simulink model "MOBATSim"  (R2020b)
settings: Solver=FixedStepAuto  StartTime=0.0  StopTime=Sim_t  FixedStep=0.01  MinStep=0.01  RelTol=1e-2
values from neighbouring files (symbols this model uses):
  Vehicles = evalin('base','Vehicles')    [I2V.m]    (also in VehicleSensors.m)
undefined symbols (not defined in the file or in its folder): Sim_Ts
libraries: simulink x50, robotalgslib x10, drivingvehiclecontroller x10, mpcadaslib x10, pid_lib x10
(part 4 of 7)

== system MOBATSim/Vehicle Model 6/Vehicle Model/Kinematic Bicycle Model ==
  v : Inport
  Steering Angle : Inport  Port=2
  Cos : Trigonometry  Operator=cos
  Gain : Gain  Gain=1/3
  Mux : Mux  Inputs=3
  Mux1 : Mux  Inputs=3
  Product : Product
  Product1 : Product
  Product2 : Product
  Saturation : Saturate  UpperLimit=pi/4  LowerLimit=-pi/4
  Sin : Trigonometry
  Tan : Trigonometry  Operator=tan
  theta : Integrator  InitialCondition=Vehicles(Vehicle_id).dynamics.orientation(4)
  x : Integrator  InitialCondition=Vehicles(Vehicle_id).dynamics.position(1)
  y : Integrator  InitialCondition=-Vehicles(Vehicle_id).dynamics.position(3)
  state : Outport
  stateDot : Outport  Port=2
  wires:
  Tan/1 -> Product2/2
  Product1/1 -> Mux1/2, y/1
  theta/1 -> Cos/1, Sin/1, Mux/3
  v/1 -> Gain/1, Product1/1, Product/1
  Gain/1 -> Product2/1
  Product/1 -> Mux1/1, x/1
  Mux/1 -> state/1
  Sin/1 -> Product1/2
  Steering Angle/1 -> Saturation/1
  Cos/1 -> Product/2
  Product2/1 -> Mux1/3, theta/1
  y/1 -> Mux/2
  x/1 -> Mux/1
  Mux1/1 -> stateDot/1
  Saturation/1 -> Tan/1

== system MOBATSim/Vehicle Model 7/Longitudinal and Lateral Controllers/Lateral Motion Control ==
  note: 1) Add Subsystem or Model blocks as valid variant choices.
      | 2) You cannot connect blocks at this level. At simulation, connectivity is automatically
      | determined, based on the active variant and port name matching.
  speed : Inport
  pose : Inport  Port=2
  changeLane : Inport  Port=3
  Pure Pursuit : Subsystem  VariantControl=PURE_PURSUIT
  Stanley : Subsystem  VariantControl=STANLEY
  SteerCmd : Outport

== system MOBATSim/Vehicle Model 7/Longitudinal and Lateral Controllers/Longitudinal Speed Control ==
  note: The vehicle calculates the speed difference between the actual speed and the reference speed, then generates the acceleration command accordingly.
  Speed Reference : Inport
  Inter Vehicular Distance : Inport  Port=2
  Lead Speed : Inport  Port=3
  Driving Mode : Inport  Port=4
  Dist2Stop : Inport  Port=5
  Actual Speed : Inport  Port=6
  Distance to Stop Controller1 : Subsystem
  Longitudinal Distance Control : Subsystem  Variant=on  VariantControlMode=label  LabelModeActiveChoice=MPC-based  mask{VehicleFollowingControl=MPC-based}
      mask prompts: VehicleFollowingControl "Vehicle Following Control"
      mask TypeOptions VehicleFollowingControl: PID-based | MPC-based
      mask Callback VehicleFollowingControl: set_param(gcb,'OverrideUsingVariant',get_param(gcb,'VehicleFollowingControl'));
      mask Display: image('MOBATSIM-Icon-Set-11 - Platoon.png'); % Use "Edit Image" on toolstrip to change.
  Reference Acceleration Generation : Subsystem
  Reference speed according to the driving mode : Subsystem
  Signal Specification1 : SignalSpecification  Dimensions=1
  Sum13 : Sum  Inputs=|+-
  Longitduinal Acceleration Command : Outport  VectorParamsAs1DForOutWhenUnconnected=off
  wires:
  Longitudinal Distance Control/1(Reference Speed) -> Reference speed according to the driving mode/3(2)
  Lead Speed/1 -> Longitudinal Distance Control/2(Lead Speed)
  Driving Mode/1 -> Reference Acceleration Generation/1(Driving Mode), Reference speed according to the driving mode/1(Driving Mode)
  Signal Specification1/1 -> Longitduinal Acceleration Command/1
  Sum13/1 -> Reference Acceleration Generation/2(Speed Error)
  Inter Vehicular Distance/1 -> Longitudinal Distance Control/1(Relative distance)
  Dist2Stop/1 -> Distance to Stop Controller1/1(Distance to Stop)
  Speed Reference/1 -> Reference speed according to the driving mode/2(1)
  Distance to Stop Controller1/1(ref speed) -> Reference speed according to the driving mode/4(4)
  Reference Acceleration Generation/1(Reference Acceleration Command) -> Signal Specification1/1
  Actual Speed/1 -> Longitudinal Distance Control/3(Ego Speed), Reference Acceleration Generation/3(Actual Speed), Sum13/2
  Reference speed according to the driving mode/1(Reference Speed) -> Sum13/1

== system MOBATSim/Vehicle Model 7/Path Planner/Astar ==
  CommunicationIDs : Inport
  Path Planner - AStar : MATLABSystem  System=VehiclePathPlanner_Astar  Vehicle_id=Vehicle_id  SimulateUsing=Interpreted execution
      mask Type: VehiclePathPlanner_Astar
      mask Display:
      | image('MOBATSIM-Icon-Set_8- Navigation.png');
      | port_label('input',1,'CommunicationIDs');
      | port_label('output',1,'waypointReached');
  waypointReached : Outport
  wires:
  CommunicationIDs/1 -> Path Planner - AStar/1
  Path Planner - AStar/1 -> waypointReached/1

== system MOBATSim/Vehicle Model 7/Path Planner/ShortestPathFinder ==
  CommunicationIDs : Inport
  Path Planner - Shortest : MATLABSystem  System=VehiclePathPlanner_shortestPathFinder  Vehicle_id=Vehicle_id  SimulateUsing=Interpreted execution
      mask Type: VehiclePathPlanner_shortestPathFinder
      mask Display:
      | image('MOBATSIM-Icon-Set_8- Navigation.png');
      | port_label('input',1,'CommunicationIDs');
      | port_label('output',1,'waypointReached');
  waypointReached : Outport
  wires:
  Path Planner - Shortest/1 -> waypointReached/1
  CommunicationIDs/1 -> Path Planner - Shortest/1

== system MOBATSim/Vehicle Model 7/Vehicle Model/Kinematic Bicycle Model ==
  v : Inport
  Steering Angle : Inport  Port=2
  Cos : Trigonometry  Operator=cos
  Gain : Gain  Gain=1/3
  Mux : Mux  Inputs=3
  Mux1 : Mux  Inputs=3
  Product : Product
  Product1 : Product
  Product2 : Product
  Saturation : Saturate  UpperLimit=pi/4  LowerLimit=-pi/4
  Sin : Trigonometry
  Tan : Trigonometry  Operator=tan
  theta : Integrator  InitialCondition=Vehicles(Vehicle_id).dynamics.orientation(4)
  x : Integrator  InitialCondition=Vehicles(Vehicle_id).dynamics.position(1)
  y : Integrator  InitialCondition=-Vehicles(Vehicle_id).dynamics.position(3)
  state : Outport
  stateDot : Outport  Port=2
  wires:
  Tan/1 -> Product2/2
  Product1/1 -> Mux1/2, y/1
  theta/1 -> Cos/1, Sin/1, Mux/3
  v/1 -> Gain/1, Product1/1, Product/1
  Gain/1 -> Product2/1
  Product/1 -> Mux1/1, x/1
  Mux/1 -> state/1
  Sin/1 -> Product1/2
  Steering Angle/1 -> Saturation/1
  Cos/1 -> Product/2
  Product2/1 -> Mux1/3, theta/1
  y/1 -> Mux/2
  x/1 -> Mux/1
  Mux1/1 -> stateDot/1
  Saturation/1 -> Tan/1

== system MOBATSim/Vehicle Model 8/Longitudinal and Lateral Controllers/Lateral Motion Control ==
  note: 1) Add Subsystem or Model blocks as valid variant choices.
      | 2) You cannot connect blocks at this level. At simulation, connectivity is automatically
      | determined, based on the active variant and port name matching.
  speed : Inport
  pose : Inport  Port=2
  changeLane : Inport  Port=3
  Pure Pursuit : Subsystem  VariantControl=PURE_PURSUIT
  Stanley : Subsystem  VariantControl=STANLEY
  SteerCmd : Outport

== system MOBATSim/Vehicle Model 8/Longitudinal and Lateral Controllers/Longitudinal Speed Control ==
  note: The vehicle calculates the speed difference between the actual speed and the reference speed, then generates the acceleration command accordingly.
  Speed Reference : Inport
  Inter Vehicular Distance : Inport  Port=2
  Lead Speed : Inport  Port=3
  Driving Mode : Inport  Port=4
  Dist2Stop : Inport  Port=5
  Actual Speed : Inport  Port=6
  Distance to Stop Controller1 : Subsystem
  Longitudinal Distance Control : Subsystem  Variant=on  VariantControlMode=label  LabelModeActiveChoice=MPC-based  mask{VehicleFollowingControl=MPC-based}
      mask prompts: VehicleFollowingControl "Vehicle Following Control"
      mask TypeOptions VehicleFollowingControl: PID-based | MPC-based
      mask Callback VehicleFollowingControl: set_param(gcb,'OverrideUsingVariant',get_param(gcb,'VehicleFollowingControl'));
      mask Display: image('MOBATSIM-Icon-Set-11 - Platoon.png'); % Use "Edit Image" on toolstrip to change.
  Reference Acceleration Generation : Subsystem
  Reference speed according to the driving mode : Subsystem
  Signal Specification1 : SignalSpecification  Dimensions=1
  Sum13 : Sum  Inputs=|+-
  Longitduinal Acceleration Command : Outport  VectorParamsAs1DForOutWhenUnconnected=off
  wires:
  Longitudinal Distance Control/1(Reference Speed) -> Reference speed according to the driving mode/3(2)
  Lead Speed/1 -> Longitudinal Distance Control/2(Lead Speed)
  Driving Mode/1 -> Reference Acceleration Generation/1(Driving Mode), Reference speed according to the driving mode/1(Driving Mode)
  Signal Specification1/1 -> Longitduinal Acceleration Command/1
  Sum13/1 -> Reference Acceleration Generation/2(Speed Error)
  Inter Vehicular Distance/1 -> Longitudinal Distance Control/1(Relative distance)
  Dist2Stop/1 -> Distance to Stop Controller1/1(Distance to Stop)
  Speed Reference/1 -> Reference speed according to the driving mode/2(1)
  Distance to Stop Controller1/1(ref speed) -> Reference speed according to the driving mode/4(4)
  Reference Acceleration Generation/1(Reference Acceleration Command) -> Signal Specification1/1
  Actual Speed/1 -> Longitudinal Distance Control/3(Ego Speed), Reference Acceleration Generation/3(Actual Speed), Sum13/2
  Reference speed according to the driving mode/1(Reference Speed) -> Sum13/1

== system MOBATSim/Vehicle Model 8/Path Planner/Astar ==
  CommunicationIDs : Inport
  Path Planner - AStar : MATLABSystem  System=VehiclePathPlanner_Astar  Vehicle_id=Vehicle_id  SimulateUsing=Interpreted execution
      mask Type: VehiclePathPlanner_Astar
      mask Display:
      | image('MOBATSIM-Icon-Set_8- Navigation.png');
      | port_label('input',1,'CommunicationIDs');
      | port_label('output',1,'waypointReached');
  waypointReached : Outport
  wires:
  CommunicationIDs/1 -> Path Planner - AStar/1
  Path Planner - AStar/1 -> waypointReached/1

== system MOBATSim/Vehicle Model 8/Path Planner/ShortestPathFinder ==
  CommunicationIDs : Inport
  Path Planner - Shortest : MATLABSystem  System=VehiclePathPlanner_shortestPathFinder  Vehicle_id=Vehicle_id  SimulateUsing=Interpreted execution
      mask Type: VehiclePathPlanner_shortestPathFinder
      mask Display:
      | image('MOBATSIM-Icon-Set_8- Navigation.png');
      | port_label('input',1,'CommunicationIDs');
      | port_label('output',1,'waypointReached');
  waypointReached : Outport
  wires:
  Path Planner - Shortest/1 -> waypointReached/1
  CommunicationIDs/1 -> Path Planner - Shortest/1

== system MOBATSim/Vehicle Model 8/Vehicle Model/Kinematic Bicycle Model ==
  v : Inport
  Steering Angle : Inport  Port=2
  Cos : Trigonometry  Operator=cos
  Gain : Gain  Gain=1/3
  Mux : Mux  Inputs=3
  Mux1 : Mux  Inputs=3
  Product : Product
  Product1 : Product
  Product2 : Product
  Saturation : Saturate  UpperLimit=pi/4  LowerLimit=-pi/4
  Sin : Trigonometry
  Tan : Trigonometry  Operator=tan
  theta : Integrator  InitialCondition=Vehicles(Vehicle_id).dynamics.orientation(4)
  x : Integrator  InitialCondition=Vehicles(Vehicle_id).dynamics.position(1)
  y : Integrator  InitialCondition=-Vehicles(Vehicle_id).dynamics.position(3)
  state : Outport
  stateDot : Outport  Port=2
  wires:
  Tan/1 -> Product2/2
  Product1/1 -> Mux1/2, y/1
  theta/1 -> Cos/1, Sin/1, Mux/3
  v/1 -> Gain/1, Product1/1, Product/1
  Gain/1 -> Product2/1
  Product/1 -> Mux1/1, x/1
  Mux/1 -> state/1
  Sin/1 -> Product1/2
  Steering Angle/1 -> Saturation/1
  Cos/1 -> Product/2
  Product2/1 -> Mux1/3, theta/1
  y/1 -> Mux/2
  x/1 -> Mux/1
  Mux1/1 -> stateDot/1
  Saturation/1 -> Tan/1

== system MOBATSim/Vehicle Model 9/Longitudinal and Lateral Controllers/Lateral Motion Control ==
  note: 1) Add Subsystem or Model blocks as valid variant choices.
      | 2) You cannot connect blocks at this level. At simulation, connectivity is automatically
      | determined, based on the active variant and port name matching.
  speed : Inport
  pose : Inport  Port=2
  changeLane : Inport  Port=3
  Pure Pursuit : Subsystem  VariantControl=PURE_PURSUIT
  Stanley : Subsystem  VariantControl=STANLEY
  SteerCmd : Outport

== system MOBATSim/Vehicle Model 9/Longitudinal and Lateral Controllers/Longitudinal Speed Control ==
  note: The vehicle calculates the speed difference between the actual speed and the reference speed, then generates the acceleration command accordingly.
  Speed Reference : Inport
  Inter Vehicular Distance : Inport  Port=2
  Lead Speed : Inport  Port=3
  Driving Mode : Inport  Port=4
  Dist2Stop : Inport  Port=5
  Actual Speed : Inport  Port=6
  Distance to Stop Controller1 : Subsystem
  Longitudinal Distance Control : Subsystem  Variant=on  VariantControlMode=label  LabelModeActiveChoice=MPC-based  mask{VehicleFollowingControl=MPC-based}
      mask prompts: VehicleFollowingControl "Vehicle Following Control"
      mask TypeOptions VehicleFollowingControl: PID-based | MPC-based
      mask Callback VehicleFollowingControl: set_param(gcb,'OverrideUsingVariant',get_param(gcb,'VehicleFollowingControl'));
      mask Display: image('MOBATSIM-Icon-Set-11 - Platoon.png'); % Use "Edit Image" on toolstrip to change.
  Reference Acceleration Generation : Subsystem
  Reference speed according to the driving mode : Subsystem
  Signal Specification1 : SignalSpecification  Dimensions=1
  Sum13 : Sum  Inputs=|+-
  Longitduinal Acceleration Command : Outport  VectorParamsAs1DForOutWhenUnconnected=off
  wires:
  Longitudinal Distance Control/1(Reference Speed) -> Reference speed according to the driving mode/3(2)
  Lead Speed/1 -> Longitudinal Distance Control/2(Lead Speed)
  Driving Mode/1 -> Reference Acceleration Generation/1(Driving Mode), Reference speed according to the driving mode/1(Driving Mode)
  Signal Specification1/1 -> Longitduinal Acceleration Command/1
  Sum13/1 -> Reference Acceleration Generation/2(Speed Error)
  Inter Vehicular Distance/1 -> Longitudinal Distance Control/1(Relative distance)
  Dist2Stop/1 -> Distance to Stop Controller1/1(Distance to Stop)
  Speed Reference/1 -> Reference speed according to the driving mode/2(1)
  Distance to Stop Controller1/1(ref speed) -> Reference speed according to the driving mode/4(4)
  Reference Acceleration Generation/1(Reference Acceleration Command) -> Signal Specification1/1
  Actual Speed/1 -> Longitudinal Distance Control/3(Ego Speed), Reference Acceleration Generation/3(Actual Speed), Sum13/2
  Reference speed according to the driving mode/1(Reference Speed) -> Sum13/1

== system MOBATSim/Vehicle Model 9/Path Planner/Astar ==
  CommunicationIDs : Inport
  Path Planner - AStar : MATLABSystem  System=VehiclePathPlanner_Astar  Vehicle_id=Vehicle_id  SimulateUsing=Interpreted execution
      mask Type: VehiclePathPlanner_Astar
      mask Display:
      | image('MOBATSIM-Icon-Set_8- Navigation.png');
      | port_label('input',1,'CommunicationIDs');
      | port_label('output',1,'waypointReached');
  waypointReached : Outport
  wires:
  CommunicationIDs/1 -> Path Planner - AStar/1
  Path Planner - AStar/1 -> waypointReached/1

== system MOBATSim/Vehicle Model 9/Path Planner/ShortestPathFinder ==
  CommunicationIDs : Inport
  Path Planner - Shortest : MATLABSystem  System=VehiclePathPlanner_shortestPathFinder  Vehicle_id=Vehicle_id  SimulateUsing=Interpreted execution
      mask Type: VehiclePathPlanner_shortestPathFinder
      mask Display:
      | image('MOBATSIM-Icon-Set_8- Navigation.png');
      | port_label('input',1,'CommunicationIDs');
      | port_label('output',1,'waypointReached');
  waypointReached : Outport
  wires:
  Path Planner - Shortest/1 -> waypointReached/1
  CommunicationIDs/1 -> Path Planner - Shortest/1

== system MOBATSim/Vehicle Model 9/Vehicle Model/Kinematic Bicycle Model ==
  v : Inport
  Steering Angle : Inport  Port=2
  Cos : Trigonometry  Operator=cos
  Gain : Gain  Gain=1/3
  Mux : Mux  Inputs=3
  Mux1 : Mux  Inputs=3
  Product : Product
  Product1 : Product
  Product2 : Product
  Saturation : Saturate  UpperLimit=pi/4  LowerLimit=-pi/4
  Sin : Trigonometry
  Tan : Trigonometry  Operator=tan
  theta : Integrator  InitialCondition=Vehicles(Vehicle_id).dynamics.orientation(4)
  x : Integrator  InitialCondition=Vehicles(Vehicle_id).dynamics.position(1)
  y : Integrator  InitialCondition=-Vehicles(Vehicle_id).dynamics.position(3)
  state : Outport
  stateDot : Outport  Port=2
  wires:
  Tan/1 -> Product2/2
  Product1/1 -> Mux1/2, y/1
  theta/1 -> Cos/1, Sin/1, Mux/3
  v/1 -> Gain/1, Product1/1, Product/1
  Gain/1 -> Product2/1
  Product/1 -> Mux1/1, x/1
  Mux/1 -> state/1
  Sin/1 -> Product1/2
  Steering Angle/1 -> Saturation/1
  Cos/1 -> Product/2
  Product2/1 -> Mux1/3, theta/1
  y/1 -> Mux/2
  x/1 -> Mux/1
  Mux1/1 -> stateDot/1
  Saturation/1 -> Tan/1

== system MOBATSim/Vehicle Model 1/Longitudinal and Lateral Controllers/Lateral Motion Control/Pure Pursuit ==
  pose : Inport
  speed : Inport  Port=2
  changeLane : Inport  Port=3
  MATLAB System : MATLABSystem  System=PurePursuit_WPGenerator  Vehicle_id=Vehicle_id  SimulateUsing=Interpreted execution
      mask Type: PurePursuit_WPGenerator
      mask Display:
      | image('MOBATSIM-Icon-Set_9- PurePursuit WP Generator.png');
      | port_label('input',1,'pose');
      | port_label('input',2,'speed');
      | port_label('input',3,'changeLane');
      | port_label('output',1,'nextWPs');
  Pure Pursuit : robotalgslib/Pure Pursuit  DesiredLinearVelocity=Vehicles(Vehicle_id).dynamics.maxSpeed  MaxAngularVelocity=1  LookaheadDistance=6  TargetDirPort=on  SimulateUsing=Code generation
  Terminator : Terminator
  Terminator1 : Terminator
  Wheel Steering Angle Formulation : Subsystem
  SteerCmd : Outport
  wires:
  MATLAB System/1 -> Pure Pursuit/2
  pose/1 -> Pure Pursuit/1, MATLAB System/1
  speed/1 -> MATLAB System/2
  changeLane/1 -> MATLAB System/3
  Pure Pursuit/3 -> Wheel Steering Angle Formulation/1(alpha)
  Pure Pursuit/1 -> Terminator/1
  Pure Pursuit/2 -> Terminator1/1
  Wheel Steering Angle Formulation/1(referenceYawAngle) -> SteerCmd/1

== system MOBATSim/Vehicle Model 1/Longitudinal and Lateral Controllers/Lateral Motion Control/Stanley ==
  pose : Inport
  speed : Inport  Port=2
  changeLane : Inport  Port=3
  Constant5 : Constant
  Deg to Rad : Gain  Gain=pi/180
  Lateral Controller Stanley : drivingvehiclecontroller/Lateral Controller Stanley  ModelType=Kinematic bicycle model  PositionGainF=2.5  PositionGainR=2.5  YawRateGain=0.2  DelayGain=0.2  VehicleMass=1575  Lf=1.2  Lr=1.6  TireStiffness=19000  Wheelbase=3  MaxSteeringAngle=35
      settings: SourceProductBaseCode=DR
  Stanley Reference Pose Generator : MATLABSystem  System=Stanley_RefPoseGenerator  Vehicle_id=Vehicle_id  SimulateUsing=Interpreted execution
      mask Type: Stanley_RefPoseGenerator
      mask Display:
      | image('MOBATSIM-Icon-Set_10- Stanley.png');
      | port_label('input',1,'pose');
      | port_label('input',2,'speed');
      | port_label('input',3,'changeLane');
      | port_label('output',1,'poseOut');
      | port_label('output',2,'referencePose');
  SteerCmd : Outport
  wires:
  Constant5/1 -> Lateral Controller Stanley/4
  Lateral Controller Stanley/1 -> Deg to Rad/1
  changeLane/1 -> Stanley Reference Pose Generator/3
  Stanley Reference Pose Generator/1 -> Lateral Controller Stanley/2
  Stanley Reference Pose Generator/2 -> Lateral Controller Stanley/1
  pose/1 -> Stanley Reference Pose Generator/1
  speed/1 -> Lateral Controller Stanley/3, Stanley Reference Pose Generator/2
  Deg to Rad/1 -> SteerCmd/1

== system MOBATSim/Vehicle Model 1/Longitudinal and Lateral Controllers/Longitudinal Speed Control/Distance to Stop Controller1 ==
  Distance to Stop : Inport
  Compare To Constant : simulink/Logic and Bit Operations/Compare To Constant  relop=>=  const=10  OutDataTypeStr=uint8
  Gain : Gain  Gain=0.08
  Product : Product
  ref speed : Outport  VectorParamsAs1DForOutWhenUnconnected=off
  wires:
  Distance to Stop/1 -> Compare To Constant/1, Gain/1
  Gain/1 -> Product/1
  Compare To Constant/1 -> Product/2
  Product/1 -> ref speed/1

== system MOBATSim/Vehicle Model 1/Longitudinal and Lateral Controllers/Longitudinal Speed Control/Longitudinal Distance Control ==
  note: 1) Add Subsystem or Model blocks as valid variant choices.
      | 2) You cannot connect blocks at this level. At simulation, connectivity is automatically
      | determined, based on the active variant and port name matching.
  Relative distance : Inport
  Lead Speed : Inport  Port=2
  Ego Speed : Inport  Port=3
  MPC-based : Subsystem  VariantControl=MPC-based
  PID-based : Subsystem  VariantControl=PID-based
  Reference Speed : Outport

== system MOBATSim/Vehicle Model 1/Longitudinal and Lateral Controllers/Longitudinal Speed Control/Reference Acceleration Generation ==
  Driving Mode : Inport
  Speed Error : Inport  Port=2
  Actual Speed : Inport  Port=3
  Emergency Brake : Constant  Value=Vehicles(Vehicle_id).dynamics.minDeceleration
  Multiport Switch3 : MultiPortSwitch  Inputs=4
  Saturation Dynamic : simulink/Discontinuities/Saturation Dynamic  OutMin=[]  OutMax=[]  OutDataTypeStr=Inherit: Same as second input  OutDataType=fixdt(1, 16)  OutScaling=2^-10  DoSatur=off
  Simple Gear Logic : MATLAB Function  TreatAsAtomicUnit=on
  Reference Acceleration Command : Outport  VectorParamsAs1DForOutWhenUnconnected=off
  wires:
  Driving Mode/1 -> Multiport Switch3/1
  Speed Error/1 -> Saturation Dynamic/2
  Emergency Brake/1 -> Saturation Dynamic/3, Multiport Switch3/4
  Saturation Dynamic/1 -> Multiport Switch3/5, Multiport Switch3/2, Multiport Switch3/3
  Actual Speed/1 -> Simple Gear Logic/1(speed)
  Multiport Switch3/1 -> Reference Acceleration Command/1
  Simple Gear Logic/1(maxAcc) -> Saturation Dynamic/1

== system MOBATSim/Vehicle Model 1/Longitudinal and Lateral Controllers/Longitudinal Speed Control/Reference speed according to the driving mode ==
  Driving Mode : Inport
  1 : Inport  Port=2
  2 : Inport  Port=3
  4 : Inport  Port=4
  Constant1 : Constant  Value=0
  Max Speed : Saturate  UpperLimit=Vehicles(Vehicle_id).dynamics.maxSpeed  LowerLimit=-100
  Multiport Switch : MultiPortSwitch  Inputs=4
  Reference Speed : Outport
  wires:
  Constant1/1 -> Multiport Switch/4
  Multiport Switch/1 -> Max Speed/1
  Driving Mode/1 -> Multiport Switch/1
  2/1 -> Multiport Switch/3
  1/1 -> Multiport Switch/2
  Max Speed/1 -> Reference Speed/1
  4/1 -> Multiport Switch/5

== system MOBATSim/Vehicle Model 10/Longitudinal and Lateral Controllers/Lateral Motion Control/Pure Pursuit ==
  pose : Inport
  speed : Inport  Port=2
  changeLane : Inport  Port=3
  MATLAB System : MATLABSystem  System=PurePursuit_WPGenerator  Vehicle_id=Vehicle_id  SimulateUsing=Interpreted execution
      mask Type: PurePursuit_WPGenerator
      mask Display:
      | image('MOBATSIM-Icon-Set_9- PurePursuit WP Generator.png');
      | port_label('input',1,'pose');
      | port_label('input',2,'speed');
      | port_label('input',3,'changeLane');
      | port_label('output',1,'nextWPs');
  Pure Pursuit : robotalgslib/Pure Pursuit  DesiredLinearVelocity=Vehicles(Vehicle_id).dynamics.maxSpeed  MaxAngularVelocity=1  LookaheadDistance=6  TargetDirPort=on  SimulateUsing=Code generation
  Terminator : Terminator
  Terminator1 : Terminator
  Wheel Steering Angle Formulation : Subsystem
  SteerCmd : Outport
  wires:
  MATLAB System/1 -> Pure Pursuit/2
  pose/1 -> Pure Pursuit/1, MATLAB System/1
  speed/1 -> MATLAB System/2
  changeLane/1 -> MATLAB System/3
  Pure Pursuit/3 -> Wheel Steering Angle Formulation/1(alpha)
  Pure Pursuit/1 -> Terminator/1
  Pure Pursuit/2 -> Terminator1/1
  Wheel Steering Angle Formulation/1(referenceYawAngle) -> SteerCmd/1

== system MOBATSim/Vehicle Model 10/Longitudinal and Lateral Controllers/Lateral Motion Control/Stanley ==
  pose : Inport
  speed : Inport  Port=2
  changeLane : Inport  Port=3
  Constant5 : Constant
  Deg to Rad : Gain  Gain=pi/180
  Lateral Controller Stanley : drivingvehiclecontroller/Lateral Controller Stanley  ModelType=Kinematic bicycle model  PositionGainF=2.5  PositionGainR=2.5  YawRateGain=0.2  DelayGain=0.2  VehicleMass=1575  Lf=1.2  Lr=1.6  TireStiffness=19000  Wheelbase=3  MaxSteeringAngle=35
      settings: SourceProductBaseCode=DR
  Stanley Reference Pose Generator : MATLABSystem  System=Stanley_RefPoseGenerator  Vehicle_id=Vehicle_id  SimulateUsing=Interpreted execution
      mask Type: Stanley_RefPoseGenerator
      mask Display:
      | image('MOBATSIM-Icon-Set_10- Stanley.png');
      | port_label('input',1,'pose');
      | port_label('input',2,'speed');
      | port_label('input',3,'changeLane');
      | port_label('output',1,'poseOut');
      | port_label('output',2,'referencePose');
  SteerCmd : Outport
  wires:
  Constant5/1 -> Lateral Controller Stanley/4
  Lateral Controller Stanley/1 -> Deg to Rad/1
  changeLane/1 -> Stanley Reference Pose Generator/3
  Stanley Reference Pose Generator/1 -> Lateral Controller Stanley/2
  Stanley Reference Pose Generator/2 -> Lateral Controller Stanley/1
  pose/1 -> Stanley Reference Pose Generator/1
  speed/1 -> Lateral Controller Stanley/3, Stanley Reference Pose Generator/2
  Deg to Rad/1 -> SteerCmd/1

== system MOBATSim/Vehicle Model 10/Longitudinal and Lateral Controllers/Longitudinal Speed Control/Distance to Stop Controller1 ==
  Distance to Stop : Inport
  Compare To Constant : simulink/Logic and Bit Operations/Compare To Constant  relop=>=  const=10  OutDataTypeStr=uint8
  Gain : Gain  Gain=0.08
  Product : Product
  ref speed : Outport  VectorParamsAs1DForOutWhenUnconnected=off
  wires:
  Distance to Stop/1 -> Compare To Constant/1, Gain/1
  Gain/1 -> Product/1
  Compare To Constant/1 -> Product/2
  Product/1 -> ref speed/1

== system MOBATSim/Vehicle Model 10/Longitudinal and Lateral Controllers/Longitudinal Speed Control/Longitudinal Distance Control ==
  note: 1) Add Subsystem or Model blocks as valid variant choices.
      | 2) You cannot connect blocks at this level. At simulation, connectivity is automatically
      | determined, based on the active variant and port name matching.
  Relative distance : Inport
  Lead Speed : Inport  Port=2
  Ego Speed : Inport  Port=3
  MPC-based : Subsystem  VariantControl=MPC-based
  PID-based : Subsystem  VariantControl=PID-based
  Reference Speed : Outport

== system MOBATSim/Vehicle Model 10/Longitudinal and Lateral Controllers/Longitudinal Speed Control/Reference Acceleration Generation ==
  Driving Mode : Inport
  Speed Error : Inport  Port=2
  Actual Speed : Inport  Port=3
  Emergency Brake : Constant  Value=Vehicles(Vehicle_id).dynamics.minDeceleration
  Multiport Switch3 : MultiPortSwitch  Inputs=4
  Saturation Dynamic : simulink/Discontinuities/Saturation Dynamic  OutMin=[]  OutMax=[]  OutDataTypeStr=Inherit: Same as second input  OutDataType=fixdt(1, 16)  OutScaling=2^-10  DoSatur=off
  Simple Gear Logic : MATLAB Function  TreatAsAtomicUnit=on
  Reference Acceleration Command : Outport  VectorParamsAs1DForOutWhenUnconnected=off
  wires:
  Driving Mode/1 -> Multiport Switch3/1
  Speed Error/1 -> Saturation Dynamic/2
  Emergency Brake/1 -> Saturation Dynamic/3, Multiport Switch3/4
  Saturation Dynamic/1 -> Multiport Switch3/5, Multiport Switch3/2, Multiport Switch3/3
  Actual Speed/1 -> Simple Gear Logic/1(speed)
  Multiport Switch3/1 -> Reference Acceleration Command/1
  Simple Gear Logic/1(maxAcc) -> Saturation Dynamic/1

== system MOBATSim/Vehicle Model 10/Longitudinal and Lateral Controllers/Longitudinal Speed Control/Reference speed according to the driving mode ==
  Driving Mode : Inport
  1 : Inport  Port=2
  2 : Inport  Port=3
  4 : Inport  Port=4
  Constant1 : Constant  Value=0
  Max Speed : Saturate  UpperLimit=Vehicles(Vehicle_id).dynamics.maxSpeed  LowerLimit=-100
  Multiport Switch : MultiPortSwitch  Inputs=4
  Reference Speed : Outport
  wires:
  Constant1/1 -> Multiport Switch/4
  Multiport Switch/1 -> Max Speed/1
  Driving Mode/1 -> Multiport Switch/1
  2/1 -> Multiport Switch/3
  1/1 -> Multiport Switch/2
  Max Speed/1 -> Reference Speed/1
  4/1 -> Multiport Switch/5

== system MOBATSim/Vehicle Model 2/Longitudinal and Lateral Controllers/Lateral Motion Control/Pure Pursuit ==
  pose : Inport
  speed : Inport  Port=2
  changeLane : Inport  Port=3
  MATLAB System : MATLABSystem  System=PurePursuit_WPGenerator  Vehicle_id=Vehicle_id  SimulateUsing=Interpreted execution
      mask Type: PurePursuit_WPGenerator
      mask Display:
      | image('MOBATSIM-Icon-Set_9- PurePursuit WP Generator.png');
      | port_label('input',1,'pose');
      | port_label('input',2,'speed');
      | port_label('input',3,'changeLane');
      | port_label('output',1,'nextWPs');
  Pure Pursuit : robotalgslib/Pure Pursuit  DesiredLinearVelocity=Vehicles(Vehicle_id).dynamics.maxSpeed  MaxAngularVelocity=1  LookaheadDistance=6  TargetDirPort=on  SimulateUsing=Code generation
  Target direction to steering angle command : Subsystem
  Terminator : Terminator
  Terminator1 : Terminator
  SteerCmd : Outport
  wires:
  MATLAB System/1 -> Pure Pursuit/2
  pose/1 -> Pure Pursuit/1, MATLAB System/1
  speed/1 -> MATLAB System/2
  changeLane/1 -> MATLAB System/3
  Pure Pursuit/3 -> Target direction to steering angle command/1(alpha)
  Pure Pursuit/1 -> Terminator/1
  Pure Pursuit/2 -> Terminator1/1
  Target direction to steering angle command/1(Ref Steering Angle) -> SteerCmd/1

== system MOBATSim/Vehicle Model 2/Longitudinal and Lateral Controllers/Lateral Motion Control/Stanley ==
  pose : Inport
  speed : Inport  Port=2
  changeLane : Inport  Port=3
  Constant5 : Constant
  Deg to Rad : Gain  Gain=pi/180
  Lateral Controller Stanley : drivingvehiclecontroller/Lateral Controller Stanley  ModelType=Kinematic bicycle model  PositionGainF=2.5  PositionGainR=2.5  YawRateGain=0.2  DelayGain=0.2  VehicleMass=1575  Lf=1.2  Lr=1.6  TireStiffness=19000  Wheelbase=3  MaxSteeringAngle=35
      settings: SourceProductBaseCode=DR
  Stanley Reference Pose Generator : MATLABSystem  System=Stanley_RefPoseGenerator  Vehicle_id=Vehicle_id  SimulateUsing=Interpreted execution
      mask Type: Stanley_RefPoseGenerator
      mask Display:
      | image('MOBATSIM-Icon-Set_10- Stanley.png');
      | port_label('input',1,'pose');
      | port_label('input',2,'speed');
      | port_label('input',3,'changeLane');
      | port_label('output',1,'poseOut');
      | port_label('output',2,'referencePose');
  SteerCmd : Outport
  wires:
  Constant5/1 -> Lateral Controller Stanley/4
  Lateral Controller Stanley/1 -> Deg to Rad/1
  changeLane/1 -> Stanley Reference Pose Generator/3
  Stanley Reference Pose Generator/1 -> Lateral Controller Stanley/2
  Stanley Reference Pose Generator/2 -> Lateral Controller Stanley/1
  pose/1 -> Stanley Reference Pose Generator/1
  speed/1 -> Lateral Controller Stanley/3, Stanley Reference Pose Generator/2
  Deg to Rad/1 -> SteerCmd/1

== system MOBATSim/Vehicle Model 2/Longitudinal and Lateral Controllers/Longitudinal Speed Control/Distance to Stop Controller ==
  Distance to Stop : Inport
  Compare To Constant : simulink/Logic and Bit Operations/Compare To Constant  relop=>=  const=10  OutDataTypeStr=uint8
  Gain : Gain  Gain=0.08
  Product : Product
  ref speed : Outport  VectorParamsAs1DForOutWhenUnconnected=off
  wires:
  Distance to Stop/1 -> Compare To Constant/1, Gain/1
  Gain/1 -> Product/1
  Compare To Constant/1 -> Product/2
  Product/1 -> ref speed/1

== system MOBATSim/Vehicle Model 2/Longitudinal and Lateral Controllers/Longitudinal Speed Control/Longitudinal Distance Control ==
  note: 1) Add Subsystem or Model blocks as valid variant choices.
      | 2) You cannot connect blocks at this level. At simulation, connectivity is automatically
      | determined, based on the active variant and port name matching.
  Relative distance : Inport
  Lead Speed : Inport  Port=2
  Ego Speed : Inport  Port=3
  MPC-based : Subsystem  VariantControl=MPC-based
  PID-based : Subsystem  VariantControl=PID-based
  Reference Speed : Outport

== system MOBATSim/Vehicle Model 2/Longitudinal and Lateral Controllers/Longitudinal Speed Control/Reference Acceleration Generation ==
  Driving Mode : Inport
  Speed Error : Inport  Port=2
  Actual Speed : Inport  Port=3
  Constant : Constant  Value=Vehicles(Vehicle_id).dynamics.minDeceleration
  Multiport Switch3 : MultiPortSwitch  Inputs=4
  Saturation Dynamic : simulink/Discontinuities/Saturation Dynamic  OutMin=[]  OutMax=[]  OutDataTypeStr=Inherit: Same as second input  OutDataType=fixdt(1, 16)  OutScaling=2^-10  DoSatur=off
  Simple Gear Logic : MATLAB Function  TreatAsAtomicUnit=on
  Reference Acceleration Command : Outport  VectorParamsAs1DForOutWhenUnconnected=off
  wires:
  Driving Mode/1 -> Multiport Switch3/1
  Speed Error/1 -> Saturation Dynamic/2
  Constant/1 -> Saturation Dynamic/3, Multiport Switch3/4
  Saturation Dynamic/1 -> Multiport Switch3/5, Multiport Switch3/2, Multiport Switch3/3
  Actual Speed/1 -> Simple Gear Logic/1(speed)
  Multiport Switch3/1 -> Reference Acceleration Command/1
  Simple Gear Logic/1(maxAcc) -> Saturation Dynamic/1

== system MOBATSim/Vehicle Model 2/Longitudinal and Lateral Controllers/Longitudinal Speed Control/Reference speed according to the driving mode ==
  Driving Mode : Inport
  1 : Inport  Port=2
  2 : Inport  Port=3
  4 : Inport  Port=4
  Constant1 : Constant  Value=0
  Max Speed : Saturate  UpperLimit=Vehicles(Vehicle_id).dynamics.maxSpeed  LowerLimit=-100
  Multiport Switch : MultiPortSwitch  Inputs=4
  Reference Speed : Outport
  wires:
  Constant1/1 -> Multiport Switch/4
  Multiport Switch/1 -> Max Speed/1
  Driving Mode/1 -> Multiport Switch/1
  2/1 -> Multiport Switch/3
  1/1 -> Multiport Switch/2
  Max Speed/1 -> Reference Speed/1
  4/1 -> Multiport Switch/5

== system MOBATSim/Vehicle Model 3/Longitudinal and Lateral Controllers/Lateral Motion Control/Pure Pursuit ==
  pose : Inport
  speed : Inport  Port=2
  changeLane : Inport  Port=3
  MATLAB System : MATLABSystem  System=PurePursuit_WPGenerator  Vehicle_id=Vehicle_id  SimulateUsing=Interpreted execution
      mask Type: PurePursuit_WPGenerator
      mask Display:
      | image('MOBATSIM-Icon-Set_9- PurePursuit WP Generator.png');
      | port_label('input',1,'pose');
      | port_label('input',2,'speed');
      | port_label('input',3,'changeLane');
      | port_label('output',1,'nextWPs');
  Pure Pursuit : robotalgslib/Pure Pursuit  DesiredLinearVelocity=Vehicles(Vehicle_id).dynamics.maxSpeed  MaxAngularVelocity=1  LookaheadDistance=6  TargetDirPort=on  SimulateUsing=Code generation
  Terminator : Terminator
  Terminator1 : Terminator
  Wheel Steering Angle Formulation : Subsystem
  SteerCmd : Outport
  wires:
  MATLAB System/1 -> Pure Pursuit/2
  pose/1 -> Pure Pursuit/1, MATLAB System/1
  speed/1 -> MATLAB System/2
  changeLane/1 -> MATLAB System/3
  Pure Pursuit/3 -> Wheel Steering Angle Formulation/1(alpha)
  Pure Pursuit/1 -> Terminator/1
  Pure Pursuit/2 -> Terminator1/1
  Wheel Steering Angle Formulation/1(referenceYawAngle) -> SteerCmd/1

== system MOBATSim/Vehicle Model 3/Longitudinal and Lateral Controllers/Lateral Motion Control/Stanley ==
  pose : Inport
  speed : Inport  Port=2
  changeLane : Inport  Port=3
  Constant5 : Constant
  Deg to Rad : Gain  Gain=pi/180
  Lateral Controller Stanley : drivingvehiclecontroller/Lateral Controller Stanley  ModelType=Kinematic bicycle model  PositionGainF=2.5  PositionGainR=2.5  YawRateGain=0.2  DelayGain=0.2  VehicleMass=1575  Lf=1.2  Lr=1.6  TireStiffness=19000  Wheelbase=3  MaxSteeringAngle=35
      settings: SourceProductBaseCode=DR
  Stanley Reference Pose Generator : MATLABSystem  System=Stanley_RefPoseGenerator  Vehicle_id=Vehicle_id  SimulateUsing=Interpreted execution
      mask Type: Stanley_RefPoseGenerator
      mask Display:
      | image('MOBATSIM-Icon-Set_10- Stanley.png');
      | port_label('input',1,'pose');
      | port_label('input',2,'speed');
      | port_label('input',3,'changeLane');
      | port_label('output',1,'poseOut');
      | port_label('output',2,'referencePose');
  SteerCmd : Outport
  wires:
  Constant5/1 -> Lateral Controller Stanley/4
  Lateral Controller Stanley/1 -> Deg to Rad/1
  changeLane/1 -> Stanley Reference Pose Generator/3
  Stanley Reference Pose Generator/1 -> Lateral Controller Stanley/2
  Stanley Reference Pose Generator/2 -> Lateral Controller Stanley/1
  pose/1 -> Stanley Reference Pose Generator/1
  speed/1 -> Lateral Controller Stanley/3, Stanley Reference Pose Generator/2
  Deg to Rad/1 -> SteerCmd/1

== system MOBATSim/Vehicle Model 3/Longitudinal and Lateral Controllers/Longitudinal Speed Control/Distance to Stop Controller1 ==
  Distance to Stop : Inport
  Compare To Constant : simulink/Logic and Bit Operations/Compare To Constant  relop=>=  const=10  OutDataTypeStr=uint8
  Gain : Gain  Gain=0.08
  Product : Product
  ref speed : Outport  VectorParamsAs1DForOutWhenUnconnected=off
  wires:
  Distance to Stop/1 -> Compare To Constant/1, Gain/1
  Gain/1 -> Product/1
  Compare To Constant/1 -> Product/2
  Product/1 -> ref speed/1

== system MOBATSim/Vehicle Model 3/Longitudinal and Lateral Controllers/Longitudinal Speed Control/Longitudinal Distance Control ==
  note: 1) Add Subsystem or Model blocks as valid variant choices.
      | 2) You cannot connect blocks at this level. At simulation, connectivity is automatically
      | determined, based on the active variant and port name matching.
  Relative distance : Inport
  Lead Speed : Inport  Port=2
  Ego Speed : Inport  Port=3
  MPC-based : Subsystem  VariantControl=MPC-based
  PID-based : Subsystem  VariantControl=PID-based
  Reference Speed : Outport

== system MOBATSim/Vehicle Model 3/Longitudinal and Lateral Controllers/Longitudinal Speed Control/Reference Acceleration Generation ==
  Driving Mode : Inport
  Speed Error : Inport  Port=2
  Actual Speed : Inport  Port=3
  Emergency Brake : Constant  Value=Vehicles(Vehicle_id).dynamics.minDeceleration
  Multiport Switch3 : MultiPortSwitch  Inputs=4
  Saturation Dynamic : simulink/Discontinuities/Saturation Dynamic  OutMin=[]  OutMax=[]  OutDataTypeStr=Inherit: Same as second input  OutDataType=fixdt(1, 16)  OutScaling=2^-10  DoSatur=off
  Simple Gear Logic : MATLAB Function  TreatAsAtomicUnit=on
  Reference Acceleration Command : Outport  VectorParamsAs1DForOutWhenUnconnected=off
  wires:
  Driving Mode/1 -> Multiport Switch3/1
  Speed Error/1 -> Saturation Dynamic/2
  Emergency Brake/1 -> Saturation Dynamic/3, Multiport Switch3/4
  Saturation Dynamic/1 -> Multiport Switch3/5, Multiport Switch3/2, Multiport Switch3/3
  Actual Speed/1 -> Simple Gear Logic/1(speed)
  Multiport Switch3/1 -> Reference Acceleration Command/1
  Simple Gear Logic/1(maxAcc) -> Saturation Dynamic/1

== system MOBATSim/Vehicle Model 3/Longitudinal and Lateral Controllers/Longitudinal Speed Control/Reference speed according to the driving mode ==
  Driving Mode : Inport
  1 : Inport  Port=2
  2 : Inport  Port=3
  4 : Inport  Port=4
  Constant1 : Constant  Value=0
  Max Speed : Saturate  UpperLimit=Vehicles(Vehicle_id).dynamics.maxSpeed  LowerLimit=-100
  Multiport Switch : MultiPortSwitch  Inputs=4
  Reference Speed : Outport
  wires:
  Constant1/1 -> Multiport Switch/4
  Multiport Switch/1 -> Max Speed/1
  Driving Mode/1 -> Multiport Switch/1
  2/1 -> Multiport Switch/3
  1/1 -> Multiport Switch/2
  Max Speed/1 -> Reference Speed/1
  4/1 -> Multiport Switch/5

== system MOBATSim/Vehicle Model 4/Longitudinal and Lateral Controllers/Lateral Motion Control/Pure Pursuit ==
  pose : Inport
  speed : Inport  Port=2
  changeLane : Inport  Port=3
  MATLAB System : MATLABSystem  System=PurePursuit_WPGenerator  Vehicle_id=Vehicle_id  SimulateUsing=Interpreted execution
      mask Type: PurePursuit_WPGenerator
      mask Display:
      | image('MOBATSIM-Icon-Set_9- PurePursuit WP Generator.png');
      | port_label('input',1,'pose');
      | port_label('input',2,'speed');
      | port_label('input',3,'changeLane');
      | port_label('output',1,'nextWPs');
  Pure Pursuit : robotalgslib/Pure Pursuit  DesiredLinearVelocity=Vehicles(Vehicle_id).dynamics.maxSpeed  MaxAngularVelocity=1  LookaheadDistance=6  TargetDirPort=on  SimulateUsing=Code generation
  Terminator : Terminator
  Terminator1 : Terminator
  Wheel Steering Angle Formulation : Subsystem
  SteerCmd : Outport
  wires:
  MATLAB System/1 -> Pure Pursuit/2
  pose/1 -> Pure Pursuit/1, MATLAB System/1
  speed/1 -> MATLAB System/2
  changeLane/1 -> MATLAB System/3
  Pure Pursuit/3 -> Wheel Steering Angle Formulation/1(alpha)
  Pure Pursuit/1 -> Terminator/1
  Pure Pursuit/2 -> Terminator1/1
  Wheel Steering Angle Formulation/1(referenceYawAngle) -> SteerCmd/1

== system MOBATSim/Vehicle Model 4/Longitudinal and Lateral Controllers/Lateral Motion Control/Stanley ==
  pose : Inport
  speed : Inport  Port=2
  changeLane : Inport  Port=3
  Constant5 : Constant
  Deg to Rad : Gain  Gain=pi/180
  Lateral Controller Stanley : drivingvehiclecontroller/Lateral Controller Stanley  ModelType=Kinematic bicycle model  PositionGainF=2.5  PositionGainR=2.5  YawRateGain=0.2  DelayGain=0.2  VehicleMass=1575  Lf=1.2  Lr=1.6  TireStiffness=19000  Wheelbase=3  MaxSteeringAngle=35
      settings: SourceProductBaseCode=DR
  Stanley Reference Pose Generator : MATLABSystem  System=Stanley_RefPoseGenerator  Vehicle_id=Vehicle_id  SimulateUsing=Interpreted execution
      mask Type: Stanley_RefPoseGenerator
      mask Display:
      | image('MOBATSIM-Icon-Set_10- Stanley.png');
      | port_label('input',1,'pose');
      | port_label('input',2,'speed');
      | port_label('input',3,'changeLane');
      | port_label('output',1,'poseOut');
      | port_label('output',2,'referencePose');
  SteerCmd : Outport
  wires:
  Constant5/1 -> Lateral Controller Stanley/4
  Lateral Controller Stanley/1 -> Deg to Rad/1
  changeLane/1 -> Stanley Reference Pose Generator/3
  Stanley Reference Pose Generator/1 -> Lateral Controller Stanley/2
  Stanley Reference Pose Generator/2 -> Lateral Controller Stanley/1
  pose/1 -> Stanley Reference Pose Generator/1
  speed/1 -> Lateral Controller Stanley/3, Stanley Reference Pose Generator/2
  Deg to Rad/1 -> SteerCmd/1

== system MOBATSim/Vehicle Model 4/Longitudinal and Lateral Controllers/Longitudinal Speed Control/Distance to Stop Controller1 ==
  Distance to Stop : Inport
  Compare To Constant : simulink/Logic and Bit Operations/Compare To Constant  relop=>=  const=10  OutDataTypeStr=uint8
  Gain : Gain  Gain=0.08
  Product : Product
  ref speed : Outport  VectorParamsAs1DForOutWhenUnconnected=off
  wires:
  Distance to Stop/1 -> Compare To Constant/1, Gain/1
  Gain/1 -> Product/1
  Compare To Constant/1 -> Product/2
  Product/1 -> ref speed/1

== system MOBATSim/Vehicle Model 4/Longitudinal and Lateral Controllers/Longitudinal Speed Control/Longitudinal Distance Control ==
  note: 1) Add Subsystem or Model blocks as valid variant choices.
      | 2) You cannot connect blocks at this level. At simulation, connectivity is automatically
      | determined, based on the active variant and port name matching.
  Relative distance : Inport
  Lead Speed : Inport  Port=2
  Ego Speed : Inport  Port=3
  MPC-based : Subsystem  VariantControl=MPC-based
  PID-based : Subsystem  VariantControl=PID-based
  Reference Speed : Outport

== system MOBATSim/Vehicle Model 4/Longitudinal and Lateral Controllers/Longitudinal Speed Control/Reference Acceleration Generation ==
  Driving Mode : Inport
  Speed Error : Inport  Port=2
  Actual Speed : Inport  Port=3
  Emergency Brake : Constant  Value=Vehicles(Vehicle_id).dynamics.minDeceleration
  Multiport Switch3 : MultiPortSwitch  Inputs=4
  Saturation Dynamic : simulink/Discontinuities/Saturation Dynamic  OutMin=[]  OutMax=[]  OutDataTypeStr=Inherit: Same as second input  OutDataType=fixdt(1, 16)  OutScaling=2^-10  DoSatur=off
  Simple Gear Logic : MATLAB Function  TreatAsAtomicUnit=on
  Reference Acceleration Command : Outport  VectorParamsAs1DForOutWhenUnconnected=off
  wires:
  Driving Mode/1 -> Multiport Switch3/1
  Speed Error/1 -> Saturation Dynamic/2
  Emergency Brake/1 -> Saturation Dynamic/3, Multiport Switch3/4
  Saturation Dynamic/1 -> Multiport Switch3/5, Multiport Switch3/2, Multiport Switch3/3
  Actual Speed/1 -> Simple Gear Logic/1(speed)
  Multiport Switch3/1 -> Reference Acceleration Command/1
  Simple Gear Logic/1(maxAcc) -> Saturation Dynamic/1

== system MOBATSim/Vehicle Model 4/Longitudinal and Lateral Controllers/Longitudinal Speed Control/Reference speed according to the driving mode ==
  Driving Mode : Inport
  1 : Inport  Port=2
  2 : Inport  Port=3
  4 : Inport  Port=4
  Constant1 : Constant  Value=0
  Max Speed : Saturate  UpperLimit=Vehicles(Vehicle_id).dynamics.maxSpeed  LowerLimit=-100
  Multiport Switch : MultiPortSwitch  Inputs=4
  Reference Speed : Outport
  wires:
  Constant1/1 -> Multiport Switch/4
  Multiport Switch/1 -> Max Speed/1
  Driving Mode/1 -> Multiport Switch/1
  2/1 -> Multiport Switch/3
  1/1 -> Multiport Switch/2
  Max Speed/1 -> Reference Speed/1
  4/1 -> Multiport Switch/5

== system MOBATSim/Vehicle Model 5/Longitudinal and Lateral Controllers/Lateral Motion Control/Pure Pursuit ==
  pose : Inport
  speed : Inport  Port=2
  changeLane : Inport  Port=3
  MATLAB System : MATLABSystem  System=PurePursuit_WPGenerator  Vehicle_id=Vehicle_id  SimulateUsing=Interpreted execution
      mask Type: PurePursuit_WPGenerator
      mask Display:
      | image('MOBATSIM-Icon-Set_9- PurePursuit WP Generator.png');
      | port_label('input',1,'pose');
      | port_label('input',2,'speed');
      | port_label('input',3,'changeLane');
      | port_label('output',1,'nextWPs');
  Pure Pursuit : robotalgslib/Pure Pursuit  DesiredLinearVelocity=Vehicles(Vehicle_id).dynamics.maxSpeed  MaxAngularVelocity=1  LookaheadDistance=6  TargetDirPort=on  SimulateUsing=Code generation
  Terminator : Terminator
  Terminator1 : Terminator
  Wheel Steering Angle Formulation : Subsystem
  SteerCmd : Outport
  wires:
  MATLAB System/1 -> Pure Pursuit/2
  pose/1 -> Pure Pursuit/1, MATLAB System/1
  speed/1 -> MATLAB System/2
  changeLane/1 -> MATLAB System/3
  Pure Pursuit/3 -> Wheel Steering Angle Formulation/1(alpha)
  Pure Pursuit/1 -> Terminator/1
  Pure Pursuit/2 -> Terminator1/1
  Wheel Steering Angle Formulation/1(referenceYawAngle) -> SteerCmd/1

== system MOBATSim/Vehicle Model 5/Longitudinal and Lateral Controllers/Lateral Motion Control/Stanley ==
  pose : Inport
  speed : Inport  Port=2
  changeLane : Inport  Port=3
  Constant5 : Constant
  Deg to Rad : Gain  Gain=pi/180
  Lateral Controller Stanley : drivingvehiclecontroller/Lateral Controller Stanley  ModelType=Kinematic bicycle model  PositionGainF=2.5  PositionGainR=2.5  YawRateGain=0.2  DelayGain=0.2  VehicleMass=1575  Lf=1.2  Lr=1.6  TireStiffness=19000  Wheelbase=3  MaxSteeringAngle=35
      settings: SourceProductBaseCode=DR
  Stanley Reference Pose Generator : MATLABSystem  System=Stanley_RefPoseGenerator  Vehicle_id=Vehicle_id  SimulateUsing=Interpreted execution
      mask Type: Stanley_RefPoseGenerator
      mask Display:
      | image('MOBATSIM-Icon-Set_10- Stanley.png');
      | port_label('input',1,'pose');
      | port_label('input',2,'speed');
      | port_label('input',3,'changeLane');
      | port_label('output',1,'poseOut');
      | port_label('output',2,'referencePose');
  SteerCmd : Outport
  wires:
  Constant5/1 -> Lateral Controller Stanley/4
  Lateral Controller Stanley/1 -> Deg to Rad/1
  changeLane/1 -> Stanley Reference Pose Generator/3
  Stanley Reference Pose Generator/1 -> Lateral Controller Stanley/2
  Stanley Reference Pose Generator/2 -> Lateral Controller Stanley/1
  pose/1 -> Stanley Reference Pose Generator/1
  speed/1 -> Lateral Controller Stanley/3, Stanley Reference Pose Generator/2
  Deg to Rad/1 -> SteerCmd/1

== system MOBATSim/Vehicle Model 5/Longitudinal and Lateral Controllers/Longitudinal Speed Control/Distance to Stop Controller1 ==
  Distance to Stop : Inport
  Compare To Constant : simulink/Logic and Bit Operations/Compare To Constant  relop=>=  const=10  OutDataTypeStr=uint8
  Gain : Gain  Gain=0.08
  Product : Product
  ref speed : Outport  VectorParamsAs1DForOutWhenUnconnected=off
  wires:
  Distance to Stop/1 -> Compare To Constant/1, Gain/1
  Gain/1 -> Product/1
  Compare To Constant/1 -> Product/2
  Product/1 -> ref speed/1

== system MOBATSim/Vehicle Model 5/Longitudinal and Lateral Controllers/Longitudinal Speed Control/Longitudinal Distance Control ==
  note: 1) Add Subsystem or Model blocks as valid variant choices.
      | 2) You cannot connect blocks at this level. At simulation, connectivity is automatically
      | determined, based on the active variant and port name matching.
  Relative distance : Inport
  Lead Speed : Inport  Port=2
  Ego Speed : Inport  Port=3
  MPC-based : Subsystem  VariantControl=MPC-based
  PID-based : Subsystem  VariantControl=PID-based
  Reference Speed : Outport
